simulink model "ldpc_encoder_580"  (R2024b)
settings: Solver=FixedStepDiscrete  StartTime=0  StopTime=0  FixedStep=1  RelTol=1e-3
model workspace (MAT data in the model file):
  G_python = [0 0 0 1 1 0 0 1 0 0 0 0 ... (668160 elements, 1152x580)]
  expected_codeword_1152 = [1 0 1 1 0 1 1 1 1 0 0 0 ... (1152 elements, 1152x1)]
  noise_mask_1152 = [0 0 0 0 0 0 0 1 0 0 0 0 ... (1152 elements, 1152x1)]
  payload_580 = [1; 0; 1; 0; 0; 1; 0; 1; 1; 0; 1; 0; 0; 1; 0; 1; 1; 0; 1; 0; 0; 1; 0; 1; 1; 0; 1; 0; 0; 1; 0; 1; 1; 0; 1; 0; 0; 0; 0; 0; 0; 0; 0; 0; 0; 0; 0; 0; 0; 0; 0; 0; 0; 0; 0; 0; 0; 0; 0; 0; 0; 0; 0; 0; 0; 0; 0; 0; 0; 0; 0; 0; 0; 0; 0; 0; 0; 0; 0; 0; 0; 0; 0; 0; 0; 0; 0; 0; 0; 0; 0; 0; 0; 0; 0; 0; 0; 0; 0; 0; 0; 0; 0; 0; 0; 0; 0; 0; 0; 0; 0; 0; 0; 0; 0; 0; 0; 0; 0; 0; 0; 0; 0; 0; 0; 0; 0; 0; 0; 0; 0; 0; 0; 0; 0; 0; 0; 0; 0; 0; 0; 0; 0; 0; 0; 0; 0; 0; 0; 0; 0; 0; 0; 0; 0; 0; 0; 0; 0; 0; 0; 0; 0; 0; 0; 0; 0; 0; 0; 0; 0; 0; 0; 0; 0; 0; 0; 0; 0; 0; 0; 0; 0; 0; 0; 0; 0; 0; 0; 0; 0; 0; 0; 0; 0; 0; 0; 0; 0; 0; 0; 0; 0; 0; 0; 0; 0; 0; 0; 0; 0; 0; 0; 0; 0; 0; 0; 0; 0; 0; 0; 0; 0; 0; 0; 0; 0; 0; 0; 0; 0; 0; 0; 0; 0; 0; 0; 0; 0; 0; 0; 0; 0; 0; 0; 0; 0; 0; 0; 0; 0; 0; 0; 0; 0; 0; 0; 0; 0; 0; 0; 0; 0; 0; 0; 0; 0; 0; 0; 0; 0; 0; 0; 0; 0; 0; 0; 0; 0; 0; 0; 0; 0; 0; 0; 0; 0; 0; 0; 0; 0; 0; 0; 0; 0; 0; 0; 0; 0; 0; 0; 0; 0; 0; 0; 0; 0; 0; 0; 0; 0; 0; 0; 0; 0; 0; 0; 0; 0; 0; 0; 0; 0; 0; 0; 0; 0; 0; 0; 0; 0; 0; 0; 0; 0; 0; 0; 0; 0; 0; 0; 0; 0; 0; 0; 0; 0; 0; 0; 0; 0; 0; 0; 0; 0; 0; 0; 0; 0; 0; 0; 0; 0; 0; 0; 0; 0; 0; 0; 0; 0; 0; 0; 0; 0; 0; 0; 0; 0; 0; 0; 0; 0; 0; 0; 0; 0; 0; 0; 0; 0; 0; 0; 0; 0; 0; 0; 0; 0; 0; 0; 0; 0; 0; 0; 0; 0; 0; 0; 0; 0; 0; 0; 0; 0; 0; 0; 0; 0; 0; 0; 0; 0; 0; 0; 0; 0; 0; 0; 0; 0; 0; 0; 0; 0; 0; 0; 0; 0; 0; 0; 0; 0; 0; 0; 0; 0; 0; 0; 0; 0; 0; 0; 0; 0; 0; 0; 0; 0; 0; 0; 0; 0; 0; 0; 0; 0; 0; 0; 0; 0; 0; 0; 0; 0; 0; 0; 0; 0; 0; 0; 0; 0; 0; 0; 0; 0; 0; 0; 0; 0; 0; 0; 0; 0; 0; 0; 0; 0; 0; 0; 0; 0; 0; 0; 0; 0; 0; 0; 0; 0; 0; 0; 0; 0; 0; 0; 0; 0; 0; 0; 0; 0; 0; 0; 0; 0; 0; 0; 0; 0; 0; 0; 0; 0; 0; 0; 0; 0; 0; 0; 0; 0; 0; 0; 0; 0; 0; 0; 0; 0; 0; 0; 0; 0; 0; 0; 0; 0; 0; 0; 0; 0; 0; 0; 0; 0; 0; 0; 0; 0; 0; 0; 0; 0; 0; 0; 0; 0; 0]
(part 1 of 2)
settings Model: Creator=HOANG AN  LastModifiedBy=HOANG AN
settings DataIOCC: SaveFormat=Array

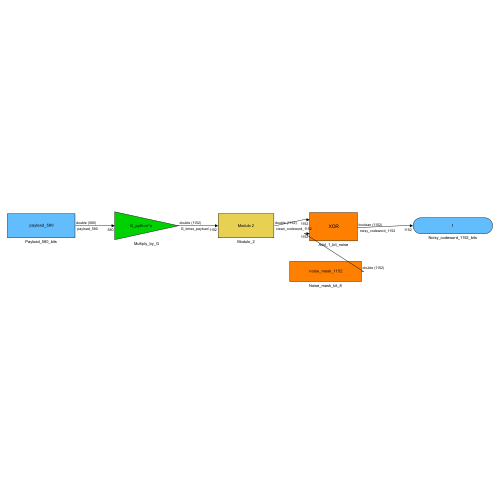
[thumbnail: Simulink's stored preview of the top-level diagram]
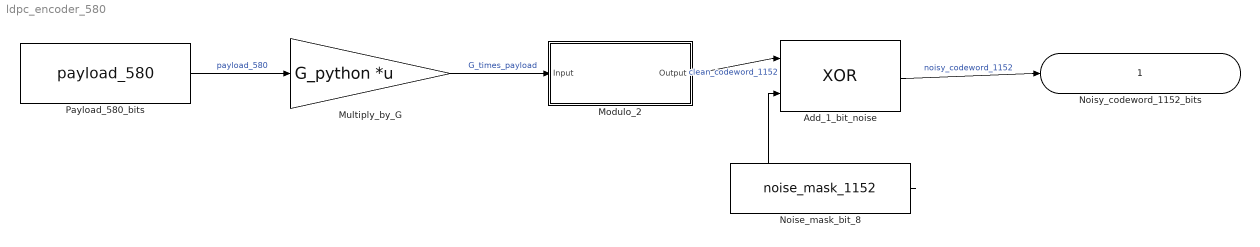
== system ldpc_encoder_580 ==
  Add_1_bit_noise : Logic  Operator=XOR  AllPortsSameDT=off  OutDataTypeStr=boolean
  Modulo_2 : Subsystem
      mask Display: disp('Modulo 2')
  Multiply_by_G : Gain  Gain=G_python  Multiplication=Matrix(K*u)
  Noise_mask_bit_8 : Constant  Value=noise_mask_1152  SampleTime=1
  Payload_580_bits : Constant  Value=payload_580  SampleTime=1
  Noisy_codeword_1152_bits : Outport
  wires:
  Payload_580_bits/1 -> Multiply_by_G/1  "payload_580"
  Multiply_by_G/1 -> Modulo_2/1(Input)  "G_times_payload"
  Modulo_2/1(Output) -> Add_1_bit_noise/1  "clean_codeword_1152"
  Noise_mask_bit_8/1 -> Add_1_bit_noise/2
  Add_1_bit_noise/1 -> Noisy_codeword_1152_bits/1  "noisy_codeword_1152"
